simulink model "untitled2I"  (R2026a)
settings: Solver=VariableStepAuto  StopTime=50  MaxStep=1e-3
values from neighbouring files (symbols this model uses):
  comdelay = 0.02    [parametro2I.m]
  Ki = block.DialogPrm(4).Data    [Ppcc2I.m]    (also in parametro2I.m = 0.1)
  Kp = block.DialogPrm(3).Data    [Ppcc2I.m]    (also in parametro2I.m = 0.5)
  pninv = 2000    [parametro2I.m]
  Ppvnom = block.DialogPrm(2).Data    [Ppcc2I.m]    (also in parametro2I.m = 10000)
  Ramp_rate_lim = block.DialogPrm(5).Data    [Ppcc2I.m]    (also in parametro2I.m = 10)
  tau_pv = 0.5    [parametro2I.m]
  tsample = block.DialogPrm(1).Data    [Ppcc2I.m]    (also in parametro2I.m = 0.2)
libraries: sl_discontinuities x5
settings Model: Creator=paulo.delgado  LastModifiedBy=paulo.delgado

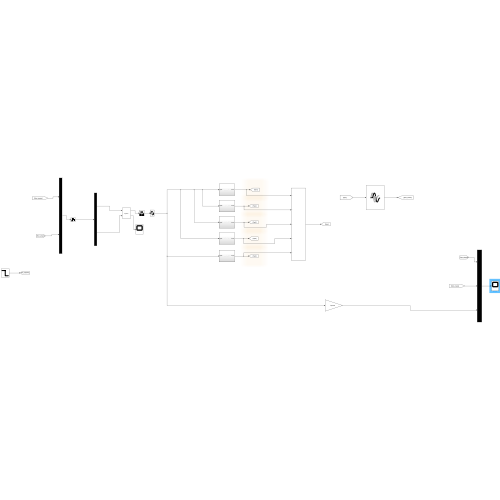
[thumbnail: Simulink's stored preview of the top-level diagram]
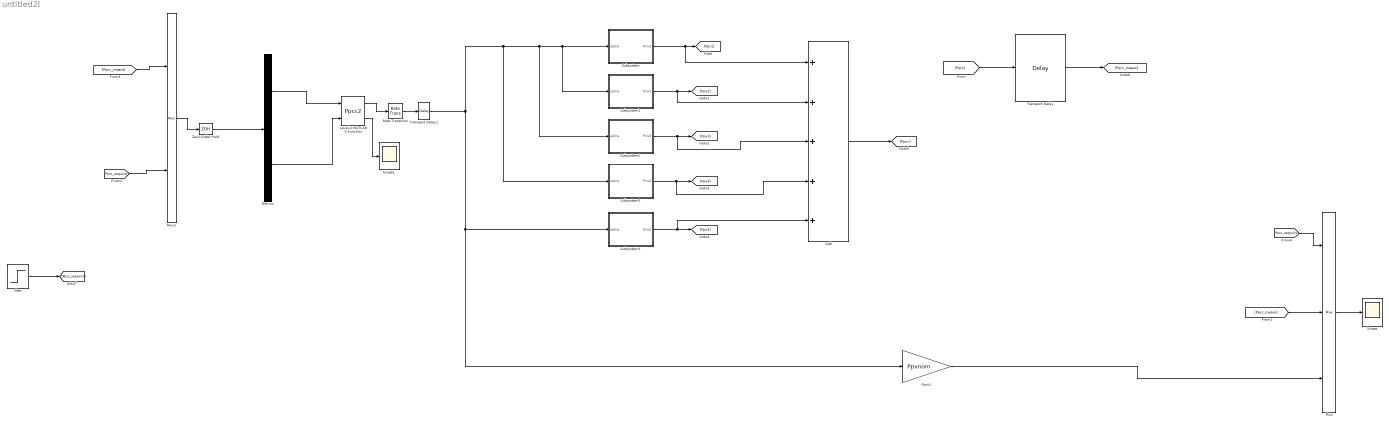
== system untitled2I ==
  Add : Sum  Inputs=+++++
  Demux : Demux  Outputs=2
  Gain1 : Gain  Gain=Ppvnom
  Level-2 MATLAB S-Function : M-S-Function  FunctionName=Ppcc2  Parameters=tsample,Ppvnom,Kp,Ki,Ramp_rate_lim
  Mux : Mux  Inputs=3
  Mux1 : Mux  Inputs=2
  Rate Transition : RateTransition  InitialCondition=7000/10000
  Scope : Scope
      settings: ActiveDisplayYMinimum=2029.591941993895  ActiveDisplayYMaximum=8592.091941993911
  Scope1 : Scope
      settings: ActiveDisplayYMinimum=9000  ActiveDisplayYMaximum=11000
  Step : Step  Time=10  InitialValue=7000  FinalValue=5000  SampleTime=0
  Subsystem : Subsystem
  Subsystem1 : Subsystem
  Subsystem2 : Subsystem
  Subsystem3 : Subsystem
  Subsystem4 : Subsystem
  Transport Delay : TransportDelay  DelayTime=comdelay  InitialOutput=7000
  Transport Delay1 : TransportDelay  DelayTime=comdelay  InitialOutput=7000/10000
  Zero-Order Hold : ZeroOrderHold  SampleTime=tsample
  wires:
  Mux/1 -> Scope/1
  Subsystem/1(Pinv1) -> Add/1, [Ppv1]
  Subsystem1/1(Pinv2) -> Add/2, [Ppv2]
  Subsystem2/1(Pinv3) -> Add/3, [Ppv3]
  Subsystem3/1(Pinv4) -> Add/4, [Ppv4]
  Subsystem4/1(Pinv5) -> Add/5, [Ppv5]
  Rate Transition/1 -> Transport Delay1/1
  Add/1 -> [Ppcc]
  [Ppcc] -> Transport Delay/1
  Transport Delay/1 -> [Ppcc_means]
  Step/1 -> [Ppcc_setpoint]
  Mux1/1 -> Zero-Order Hold/1
  Zero-Order Hold/1 -> Demux/1
  Demux/1 -> Level-2 MATLAB S-Function/1
  Demux/2 -> Level-2 MATLAB S-Function/2
  Level-2 MATLAB S-Function/1 -> Rate Transition/1
  [Ppcc_means] -> Mux1/1
  [Ppcc_setpoint] -> Mux1/2
  [Ppcc_means] -> Mux/2
  [Ppcc_setpoint] -> Mux/1
  Transport Delay1/1 -> Subsystem3/1(alpha), Subsystem2/1(alpha), Subsystem1/1(alpha), Subsystem/1(alpha), Gain1/1, Subsystem4/1(alpha)
  Level-2 MATLAB S-Function/2 -> Scope1/1
  Gain1/1 -> Mux/3

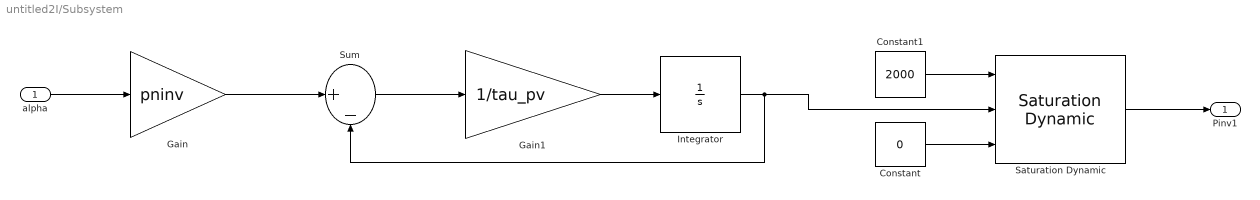
== system untitled2I/Subsystem ==
  alpha : Inport
  Constant : Constant  Value=0
  Constant1 : Constant  Value=2000
  Gain : Gain  Gain=pninv
  Gain1 : Gain  Gain=1/tau_pv
  Integrator : Integrator  InitialCondition=7000/5
  Saturation Dynamic : sl_discontinuities/Saturation Dynamic  OutMin=[]  OutMax=[]  OutDataTypeStr=Inherit: Same as second input  OutDataType=fixdt(1, 16)  OutScaling=2^-10  DoSatur=off
      settings: LibrarySourceBlock=|
      | simulink/Discontinuities/Saturation
      | Dynamic
  Sum : Sum  Inputs=|+-
  Pinv1 : Outport
  wires:
  Integrator/1 -> Saturation Dynamic/2, Sum/2
  Constant/1 -> Saturation Dynamic/3
  Sum/1 -> Gain1/1
  Gain1/1 -> Integrator/1
  Saturation Dynamic/1 -> Pinv1/1
  Gain/1 -> Sum/1
  Constant1/1 -> Saturation Dynamic/1
  alpha/1 -> Gain/1

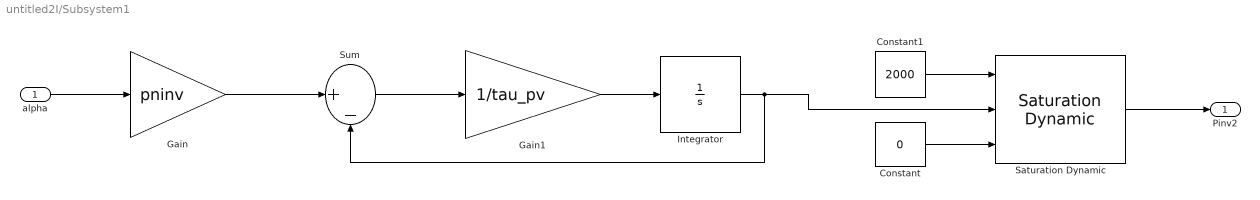
== system untitled2I/Subsystem1 ==
  alpha : Inport
  Constant : Constant  Value=0
  Constant1 : Constant  Value=2000
  Gain : Gain  Gain=pninv
  Gain1 : Gain  Gain=1/tau_pv
  Integrator : Integrator  InitialCondition=7000/5
  Saturation Dynamic : sl_discontinuities/Saturation Dynamic  OutMin=[]  OutMax=[]  OutDataTypeStr=Inherit: Same as second input  OutDataType=fixdt(1, 16)  OutScaling=2^-10  DoSatur=off
      settings: LibrarySourceBlock=|
      | simulink/Discontinuities/Saturation
      | Dynamic
  Sum : Sum  Inputs=|+-
  Pinv2 : Outport
  wires:
  alpha/1 -> Gain/1
  Constant1/1 -> Saturation Dynamic/1
  Gain/1 -> Sum/1
  Saturation Dynamic/1 -> Pinv2/1
  Gain1/1 -> Integrator/1
  Sum/1 -> Gain1/1
  Constant/1 -> Saturation Dynamic/3
  Integrator/1 -> Sum/2, Saturation Dynamic/2

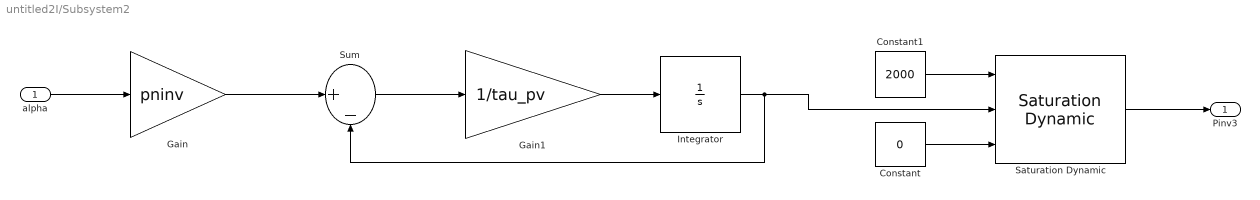
== system untitled2I/Subsystem2 ==
  alpha : Inport
  Constant : Constant  Value=0
  Constant1 : Constant  Value=2000
  Gain : Gain  Gain=pninv
  Gain1 : Gain  Gain=1/tau_pv
  Integrator : Integrator  InitialCondition=7000/5
  Saturation Dynamic : sl_discontinuities/Saturation Dynamic  OutMin=[]  OutMax=[]  OutDataTypeStr=Inherit: Same as second input  OutDataType=fixdt(1, 16)  OutScaling=2^-10  DoSatur=off
      settings: LibrarySourceBlock=|
      | simulink/Discontinuities/Saturation
      | Dynamic
  Sum : Sum  Inputs=|+-
  Pinv3 : Outport
  wires:
  Integrator/1 -> Saturation Dynamic/2, Sum/2
  Constant/1 -> Saturation Dynamic/3
  Sum/1 -> Gain1/1
  Gain1/1 -> Integrator/1
  Saturation Dynamic/1 -> Pinv3/1
  Gain/1 -> Sum/1
  Constant1/1 -> Saturation Dynamic/1
  alpha/1 -> Gain/1

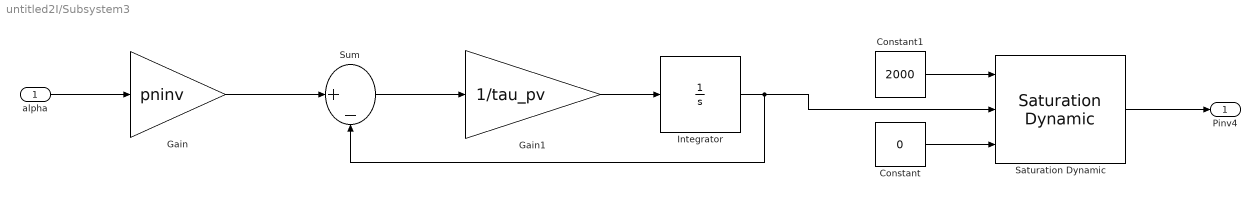
== system untitled2I/Subsystem3 ==
  alpha : Inport
  Constant : Constant  Value=0
  Constant1 : Constant  Value=2000
  Gain : Gain  Gain=pninv
  Gain1 : Gain  Gain=1/tau_pv
  Integrator : Integrator  InitialCondition=7000/5
  Saturation Dynamic : sl_discontinuities/Saturation Dynamic  OutMin=[]  OutMax=[]  OutDataTypeStr=Inherit: Same as second input  OutDataType=fixdt(1, 16)  OutScaling=2^-10  DoSatur=off
      settings: LibrarySourceBlock=|
      | simulink/Discontinuities/Saturation
      | Dynamic
  Sum : Sum  Inputs=|+-
  Pinv4 : Outport
  wires:
  alpha/1 -> Gain/1
  Constant1/1 -> Saturation Dynamic/1
  Gain/1 -> Sum/1
  Saturation Dynamic/1 -> Pinv4/1
  Gain1/1 -> Integrator/1
  Sum/1 -> Gain1/1
  Constant/1 -> Saturation Dynamic/3
  Integrator/1 -> Sum/2, Saturation Dynamic/2

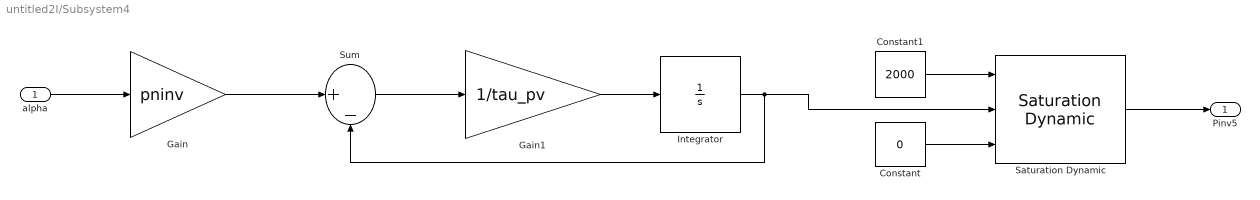
== system untitled2I/Subsystem4 ==
  alpha : Inport
  Constant : Constant  Value=0
  Constant1 : Constant  Value=2000
  Gain : Gain  Gain=pninv
  Gain1 : Gain  Gain=1/tau_pv
  Integrator : Integrator  InitialCondition=7000/5
  Saturation Dynamic : sl_discontinuities/Saturation Dynamic  OutMin=[]  OutMax=[]  OutDataTypeStr=Inherit: Same as second input  OutDataType=fixdt(1, 16)  OutScaling=2^-10  DoSatur=off
      settings: LibrarySourceBlock=|
      | simulink/Discontinuities/Saturation
      | Dynamic
  Sum : Sum  Inputs=|+-
  Pinv5 : Outport
  wires:
  Integrator/1 -> Saturation Dynamic/2, Sum/2
  Constant/1 -> Saturation Dynamic/3
  Sum/1 -> Gain1/1
  Gain1/1 -> Integrator/1
  Saturation Dynamic/1 -> Pinv5/1
  Gain/1 -> Sum/1
  Constant1/1 -> Saturation Dynamic/1
  alpha/1 -> Gain/1
